simulink model "lab3_sim"  (R2026a)
settings: Solver=VariableStepAuto  StopTime=10
values from neighbouring files (symbols this model uses):
  A = [0,              0,             w0,        0 ... (first row only)    [lab3_t3.m]    (also in lab4_m.m = [          0,            0,      omega0,           0)
  B = [0 ... (first row only)    [lab4_m.m]
  B_d = [0; 0; 0; 1/(w0*J2)]    [lab3_t3.m]
  B_I = [0; 0; kI/(w0*J1); 0]    [lab3_t3.m]
  K = place(A, B_I, desired_poles)    [lab3_t3.m]    (also in lab4_m.m = K_1_2)
undefined symbols (not defined in the file or in its folder): K_list
settings Model: Creator=yonmi

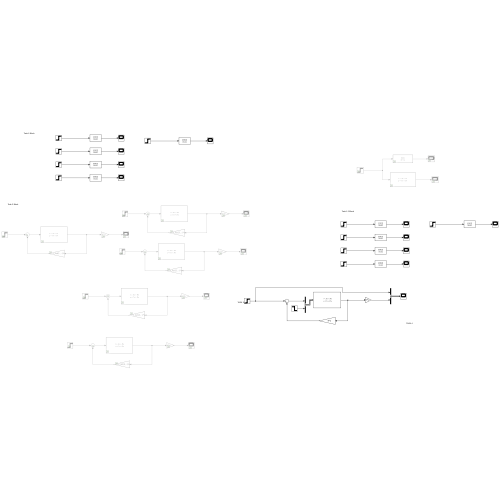
[thumbnail: Simulink's stored preview of the top-level diagram]
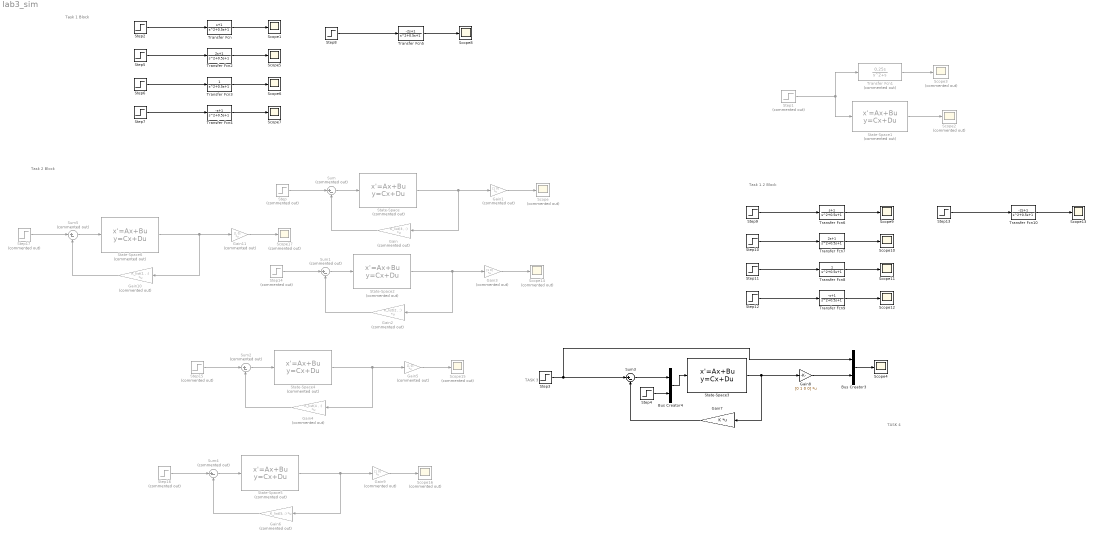
== system lab3_sim ==
  note: Task 1.2 Block
  note: Task 1 Block
  note: Task 2 Block
  note: TASK 4
  note: TASK 3
  Bus Creator3 : BusCreator  Inputs=2
  Bus Creator4 : BusCreator  Inputs=2
  Gain : Gain  Commented=on  Gain=K_list(3 , :)  Multiplication=Matrix(K*u)
  Gain{1,3,5,9,11} (5 alike) : Gain  Commented=on  Gain=[1 0]  Multiplication=Matrix(K*u)
  Gain10 : Gain  Commented=on  Gain=K_list(1 , :)  Multiplication=Matrix(K*u)
  Gain2 : Gain  Commented=on  Gain=K_list(2 , :)  Multiplication=Matrix(K*u)
  Gain4 : Gain  Commented=on  Gain=K_list(4 , :)  Multiplication=Matrix(K*u)
  Gain6 : Gain  Commented=on  Gain=K_list(5, :)  Multiplication=Matrix(K*u)
  Gain7 : Gain  Gain=K  Multiplication=Matrix(K*u)
  Gain8 : Gain  Gain=[0 1 0 0]  Multiplication=Matrix(K*u)
  Scope{,2..3,14..17} (7 alike) : Scope  Commented=on
      Scope settings: ActiveDisplayYMinimum=-0.25636925954186979  ActiveDisplayYMaximum=1.2602810485464728
      Scope14 settings: ActiveDisplayYMinimum=-0.25636925954186979  ActiveDisplayYMaximum=1.2602810485464728  DataLoggingVariableName=ScopeData14
      Scope15 settings: ActiveDisplayYMinimum=-0.25636925954186979  ActiveDisplayYMaximum=1.2602810485464728  DataLoggingVariableName=ScopeData15
      Scope16 settings: ActiveDisplayYMinimum=-0.25636925954186979  ActiveDisplayYMaximum=1.2602810485464728  DataLoggingVariableName=ScopeData16
      Scope17 settings: ActiveDisplayYMinimum=-0.25636925954186979  ActiveDisplayYMaximum=1.2602810485464728  DataLoggingVariableName=ScopeData17
      Scope2 settings: ActiveDisplayYMinimum=-0.31222  ActiveDisplayYMaximum=2.80994  DataLoggingVariableName=ScopeData2
      Scope3 settings: ActiveDisplayYMinimum=-0.31222  ActiveDisplayYMaximum=2.80994  DataLoggingVariableName=ScopeData3
  Scope{1,4..13} (11 alike) : Scope
      Scope1 settings: ActiveDisplayYMinimum=-0.21068366722933168  ActiveDisplayYMaximum=1.8961530050639857  DataLoggingVariableName=ScopeData4
      Scope10 settings: DataLoggingVariableName=ScopeData9
      Scope11 settings: DataLoggingVariableName=ScopeData10
      Scope12 settings: DataLoggingVariableName=ScopeData11
      Scope13 settings: DataLoggingVariableName=ScopeData12
      Scope4 settings: ActiveDisplayYMinimum=-0.41934000313389941  ActiveDisplayYMaximum=1.8254804043937631
      Scope5 settings: ActiveDisplayYMinimum=-0.2805519932388883  ActiveDisplayYMaximum=2.5249679391499953  DataLoggingVariableName=ScopeData5
      Scope6 settings: ActiveDisplayYMinimum=-0.18038400477599556  ActiveDisplayYMaximum=1.6234560429839604  DataLoggingVariableName=ScopeData6
      Scope7 settings: ActiveDisplayYMinimum=-0.56863310619947072  ActiveDisplayYMaximum=1.8321385675873083  DataLoggingVariableName=ScopeData7
      Scope8 settings: DataLoggingVariableName=ScopeData8
      Scope9 settings: ActiveDisplayYMinimum=-0.21068366722933168  ActiveDisplayYMaximum=1.8961530050639857  DataLoggingVariableName=ScopeData13
  State-Space{,2,4..6} (5 alike) : StateSpace  Commented=on  A=A  B=B  C=eye(2)  D=[0;0]  InitialCondition=1
  State-Space1 : StateSpace  Commented=on  A=A  B=B  C=[1 0]  D=[0]  InitialCondition=0
  State-Space3 : StateSpace  A=A  B=[B_I B_d]  C=eye(4)  D=[0 0; 0 0; 0 0;0 0 ]  InitialCondition=0
  Step{,14..17} (5 alike) : Step  Commented=on  Time=3  FinalValue=3  SampleTime=0
  Step1 : Step  Commented=on  Time=3  FinalValue=10  SampleTime=0
  Step{2..3,5..13} (11 alike) : Step  SampleTime=0
  Step4 : Step  Time=5  FinalValue=-1  SampleTime=0
  Sum{,1..2,4..5} (5 alike) : Sum  Commented=on  Inputs=|+-
  Sum3 : Sum  Inputs=|+-
  Transfer Fcn : TransferFcn  Numerator=[1 1]  Denominator=[1 0.5 1]
  Transfer Fcn1 : TransferFcn  Commented=on  Numerator=[0.25 0]  Denominator=[1 1 0]
  Transfer Fcn10 : TransferFcn  Numerator=[-2 1]  Denominator=[1 0.5 1]
  Transfer Fcn2 : TransferFcn  Numerator=[2 1]  Denominator=[1 0.5 1]
  Transfer Fcn3 : TransferFcn  Numerator=[0 1]  Denominator=[1 0.5 1]
  Transfer Fcn4 : TransferFcn  Numerator=[-1 1]  Denominator=[1 0.5 1]
  Transfer Fcn5 : TransferFcn  Numerator=[-2 1]  Denominator=[1 0.5 1]
  Transfer Fcn6 : TransferFcn  Numerator=[1 1]  Denominator=[1 0.5 1]
  Transfer Fcn7 : TransferFcn  Numerator=[2 1]  Denominator=[1 0.5 1]
  Transfer Fcn8 : TransferFcn  Numerator=[0 1]  Denominator=[1 0.5 1]
  Transfer Fcn9 : TransferFcn  Numerator=[-1 1]  Denominator=[1 0.5 1]
  wires:
  State-Space/1 -> Gain1/1, Gain/1
  Gain/1 -> Sum/2
  Sum/1 -> State-Space/1
  Step/1 -> Sum/1
  Gain1/1 -> Scope/1
  Step1/1 -> State-Space1/1, Transfer Fcn1/1
  State-Space1/1 -> Scope2/1
  Transfer Fcn1/1 -> Scope3/1
  Step4/1 -> Bus Creator4/2
  Sum3/1 -> Bus Creator4/1
  Bus Creator4/1 -> State-Space3/1
  Bus Creator3/1 -> Scope4/1
  Gain7/1 -> Sum3/2
  Step3/1 -> Sum3/1, Bus Creator3/1
  State-Space3/1 -> Gain7/1, Gain8/1
  Gain8/1 -> Bus Creator3/2
  Step2/1 -> Transfer Fcn/1
  Transfer Fcn/1 -> Scope1/1
  Transfer Fcn2/1 -> Scope5/1
  Step5/1 -> Transfer Fcn2/1
  Transfer Fcn3/1 -> Scope6/1
  Step6/1 -> Transfer Fcn3/1
  Transfer Fcn4/1 -> Scope7/1
  Step7/1 -> Transfer Fcn4/1
  Transfer Fcn5/1 -> Scope8/1
  Step8/1 -> Transfer Fcn5/1
  Transfer Fcn7/1 -> Scope10/1
  Transfer Fcn10/1 -> Scope13/1
  Transfer Fcn8/1 -> Scope11/1
  Transfer Fcn6/1 -> Scope9/1
  Step10/1 -> Transfer Fcn7/1
  Step9/1 -> Transfer Fcn6/1
  Step11/1 -> Transfer Fcn8/1
  Step13/1 -> Transfer Fcn10/1
  Transfer Fcn9/1 -> Scope12/1
  Step12/1 -> Transfer Fcn9/1
  State-Space2/1 -> Gain3/1, Gain2/1
  Sum1/1 -> State-Space2/1
  Step14/1 -> Sum1/1
  Gain2/1 -> Sum1/2
  Gain3/1 -> Scope14/1
  State-Space4/1 -> Gain5/1, Gain4/1
  Sum2/1 -> State-Space4/1
  Step15/1 -> Sum2/1
  Gain4/1 -> Sum2/2
  Gain5/1 -> Scope15/1
  State-Space5/1 -> Gain9/1, Gain6/1
  Sum4/1 -> State-Space5/1
  Step16/1 -> Sum4/1
  Gain6/1 -> Sum4/2
  Gain9/1 -> Scope16/1
  State-Space6/1 -> Gain11/1, Gain10/1
  Sum5/1 -> State-Space6/1
  Step17/1 -> Sum5/1
  Gain10/1 -> Sum5/2
  Gain11/1 -> Scope17/1
